simulink model "acf_force_control_fixed_upper_20261005"  (R2026b)
settings: Solver=ode4  StopTime=2  FixedStep=3.3333333333333333e-06
PostLoadFcn:
  | addpath(fullfile(fileparts(get_param(bdroot,'FileName')),'helpers'));
InitFcn:
  | acf_fixed_apply(bdroot);
model workspace (MAT data in the model file):
  p : object (value not decoded)
  pCompliant : object (value not decoded)
  pDefault : object (value not decoded)
symbols that are objects in the model workspace (value not decoded): p
undefined symbols (not defined in the file or in its folder): DiscIntNeverNeededParam
(part 1 of 3)
settings Model: Creator=tommie  LastModifiedBy=tommie
settings DataIOCC: SignalLogging=off
settings DebuggingCC: AlgebraicLoopMsg=error
settings RTWCC: GenCodeOnly=on
settings GRTTargetCC: MatFileLogging=off

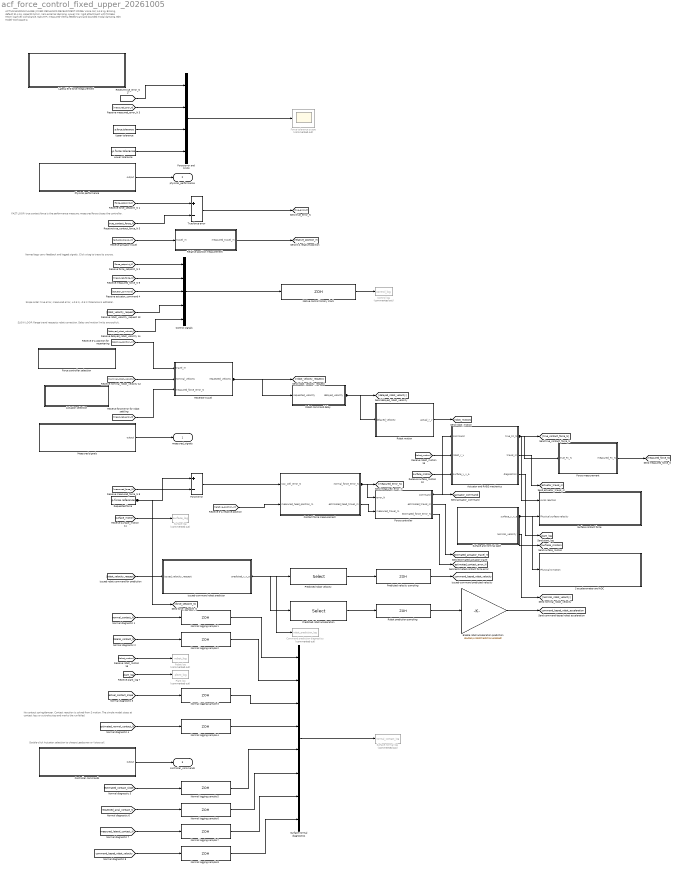
== system acf_force_control_fixed_upper_20261005 ==
  note: FAST LOOP: true contact force is the performance measure; measured force closes the controller.
  note: SLOW LOOP: flange travel requests robot correction. Delay and motion limits are explicit.
  note: No contact spring/damper. Contact reaction is solved from S motion.
      | The simple model stops at contact loss or a stroke stop and marks the run failed.
  note: Scope order: true error, measured error, +0.5 N, -0.5 N (tolerance is editable).
  note: Double-click Actuator selection to choose Leadscrew or Voice coil.
  note: Named tags carry feedback and logged signals. Click a tag to trace its source.
  note: ACTIVE SANDING FLANGE | FIXED MECHANICS DEVELOPMENT MODEL
      | Voice coil; A1.5 kg, B0.6 kg, default S1.4 kg. Upper20 N/mm, zero external damping.
      | Lower link: rigid attachment with finite64 MN/m load-cell compliance.
      | Native PI, measured-inertia feedforward and bounded modal damping. Edit Model Workspace p.
  Actuator and RABS mechanics : Subsystem
  Actuator selection : Subsystem  mask(Active contact flange actuator selection){ActuatorChoice=Voice coil}
      mask prompts: ActuatorChoice "Actuator"
      mask help: Choose the motor before running. Mechanical, surface and sensor settings are preserved. Force-controller gains, command units and initial holding current are recalculated for the selected drive.
      mask TypeOptions ActuatorChoice: Leadscrew | Voice coil | Ideal position (reference)
      mask Callback ActuatorChoice: acf_fixed_select_actuator(bdroot(gcb),get_param(gcb,'ActuatorChoice'));
      mask Display: disp(sprintf('Actuator selection\n%s',get_param(gcb,'ActuatorChoice')));
  Command prediction diagnostics : ToWorkspace  Commented=on  VariableName=robot_prediction_log  SaveFormat=Timeseries  SampleTime=p.sim.step
  Contact force measurement : Subsystem
  Control log : ToWorkspace  Commented=on  VariableName=control_log  SaveFormat=Timeseries  SampleTime=p.sim.step
  Control signals : Mux  Inputs=5
  Controller commands : Subsystem
  Enable robot acceleration prediction : Gain  Gain=double(p.robotPrediction.enabled)
  Force controller : Subsystem  Variant=on  VariantControlMode=label  LabelModeActiveChoice=Coil PI and PID
  Force controller selection : Subsystem  mask{ControllerChoice=PI, AccelerationFeedforward=on}
      mask prompts: ControllerChoice "Voice-coil control strategy"; AccelerationFeedforward "Measured acceleration feedforward"
      mask help: Native force/stroke observer or conventional force PI/PID. Gains remain editable in the Model Workspace p. The saved recommended preset includes the qualified upper-rigid PID gains.
      mask TypeOptions ControllerChoice: PI | PID
      mask Callback ControllerChoice: acf_fixed_select_controller(bdroot);
      mask Callback AccelerationFeedforward: acf_fixed_select_controller(bdroot(gcb));
      mask Display: disp('Choose coil controller')
  Force error : Sum  Inputs=+-
  Force error and limits : Mux
  Force measurement : Subsystem
  Force tolerance scope : Scope  Commented=on
  Issued-command robot predictor : Subsystem
  Lateral B-S force measurement : Subsystem
  Lower tolerance : Constant  Value=-p.force.tolerance
  Measured signals : Subsystem
  Native control history clock : ZeroOrderHold  SampleTime=p.sim.step
  Normal logging sample {1..8} (8 alike) : ZeroOrderHold  SampleTime=p.sim.step
  Physical performance : Subsystem
  Plant log : ToWorkspace  Commented=on  VariableName=plant_log  SaveFormat=Timeseries  SampleTime=p.sim.step
  Predicted robot acceleration : Selector  InputPortWidth=3  IndexOptions=Index vector (dialog)  Indices=3  OutputSizes=1
  Predicted robot velocity : Selector  InputPortWidth=3  IndexOptions=Index vector (dialog)  Indices=2  OutputSizes=1
  Predicted velocity sampling : ZeroOrderHold  SampleTime=p.force.sampleTime
  Recenter travel : Subsystem
  Relative position measurement : Subsystem
  Requested force : Constant  Value=p.force.reference
  Robot command delay : Subsystem
  Robot log : ToWorkspace  Commented=on  VariableName=robot_log  SaveFormat=Timeseries  SampleTime=p.sim.step
  Robot motion : Subsystem
  Robot prediction sampling : ZeroOrderHold  SampleTime=p.force.sampleTime
  S accelerometer and ADC : Subsystem
  Surface and nominal path : Subsystem
  Surface contact force : Subsystem
  Surface log : ToWorkspace  Commented=on  VariableName=surface_log  SaveFormat=Timeseries  SampleTime=p.sim.step
  Surface normal diagnostics : Mux  Inputs=8
  Surface normal log : ToWorkspace  Commented=on  VariableName=normal_contact_log  SaveFormat=Timeseries  SampleTime=p.sim.step
  True force error : Sum  Inputs=+-
  Upper tolerance : Constant  Value=p.force.tolerance
  measured_signals : Outport
  physical_performance : Outport  Port=2
  controller_commands : Outport  Port=3
  tag scope: command_based_robot_acceleration=global, command_based_robot_velocity=global, estimated_actuator_travel_m=global, estimated_contact_error_N=global, plant_log=global, surface_motion=global
  wires:
  Force measurement/1(measured_Fc_N) -> [measured_force_N]
  Enable robot acceleration prediction/1 -> [command_based_robot_acceleration]
  Surface and nominal path/1(surface_y_v_a) -> S accelerometer and ADC/1(Physical S motion), Surface contact force/2(Physical surface velocity), [surface_motion]
  Surface and nominal path/2(nominal_velocity) -> [nominal_robot_velocity]
  Actuator and RABS mechanics/3(diagnostics) -> [plant_log]
  Actuator and RABS mechanics/1(true_Fc_N) -> Surface contact force/1(Axial reaction), [true_contact_force_N], Force measurement/1(true_Fc_N)
  Robot prediction sampling/1 -> Enable robot acceleration prediction/1
  Predicted velocity sampling/1 -> [command_based_robot_velocity]
  Force controller/3(estimated_force_error_N) -> [estimated_contact_error_N]
  Force controller/2(estimated_travel_m) -> [estimated_actuator_travel_m]
  Controller commands/1(output) -> controller_commands/1
  [actual_contact_slope] -> Normal logging sample 3/1
  Predicted robot acceleration/1 -> Robot prediction sampling/1
  Lower tolerance/1 -> Force error and limits/4
  Force error/1 -> Contact force measurement/1(raw_cell_error_N)
  [relative_position_m] -> Contact force measurement/2(measured_head_position_m)
  [normal_contact_N] -> Normal logging sample 1/1
  [measured_force_N] -> Force error/2
  [command_based_robot_velocity] -> Normal logging sample 8/1
  [estimated_contact_slope] -> Normal logging sample 5/1
  Recenter travel/1(requested_velocity) -> [robot_velocity_request], Robot command delay/1(requested_velocity)
  Requested force/1 -> [force_setpoint_N], Force error/1
  [robot_velocity_request] -> Issued-command robot predictor/1(issued_velocity_request)
  [robot_velocity_request] -> Control signals/4
  [relative_position_m] -> Recenter travel/1(travel_m)
  [measured_error_N] -> Force error and limits/2
  [measured_lateral_contact_N] -> Normal logging sample 7/1
  Issued-command robot predictor/1(predicted_r_v_a) -> Predicted robot velocity/1, Command prediction diagnostics/1, Predicted robot acceleration/1
  [actuator_command] -> Control signals/3
  Measured signals/1(output) -> measured_signals/1
  Physical performance/1(output) -> physical_performance/1
  [estimated_normal_contact_N] -> Normal logging sample 4/1
  [plant_log] -> Plant log/1
  [measured_error_N] -> Recenter travel/3(measured_force_error_N)
  Robot command delay/1(delayed_velocity) -> [delayed_robot_velocity], Robot motion/1(delayed_velocity)
  [force_setpoint_N] -> True force error/1
  [true_error_N] -> Force error and limits/1
  Robot motion/1(actual_r_v) -> [robot_motion]
  Normal logging sample 8/1 -> Surface normal diagnostics/8
  Upper tolerance/1 -> Force error and limits/3
  [true_contact_force_N] -> True force error/2
  [surface_motion] -> Actuator and RABS mechanics/3(surface_y_v_a)
  Normal logging sample 5/1 -> Surface normal diagnostics/5
  [delayed_robot_velocity] -> Control signals/5
  [measured_force_N] -> Control signals/2
  Normal logging sample 3/1 -> Surface normal diagnostics/3
  Contact force measurement/2(estimated_head_travel_m) -> Force controller/2(measured_travel_m)
  [nominal_robot_velocity] -> Recenter travel/2(nominal_velocity)
  [requested_axial_contact_N] -> Normal logging sample 6/1
  Relative position measurement/1(measured_travel_m) -> [relative_position_m]
  Control signals/1 -> Native control history clock/1
  Force error and limits/1 -> Force tolerance scope/1
  [actuator_travel_m] -> Relative position measurement/1(travel_m)
  Force controller/1(command) -> [actuator_command], Actuator and RABS mechanics/1(command)
  True force error/1 -> [true_error_N]
  [robot_motion] -> Robot log/1
  Normal logging sample 1/1 -> Surface normal diagnostics/1
  Normal logging sample 2/1 -> Surface normal diagnostics/2
  Normal logging sample 4/1 -> Surface normal diagnostics/4
  Normal logging sample 6/1 -> Surface normal diagnostics/6
  Actuator and RABS mechanics/2(travel_m) -> [actuator_travel_m]
  Normal logging sample 7/1 -> Surface normal diagnostics/7
  [surface_motion] -> Surface log/1
  Contact force measurement/1(normal_force_error_N) -> [measured_error_N], Force controller/1(error_N)
  Predicted robot velocity/1 -> Predicted velocity sampling/1
  [lateral_contact_N] -> Normal logging sample 2/1
  Surface normal diagnostics/1 -> Surface normal log/1
  [force_setpoint_N] -> Control signals/1
  Native control history clock/1 -> Control log/1
  [robot_motion] -> Actuator and RABS mechanics/2(robot_r_v)

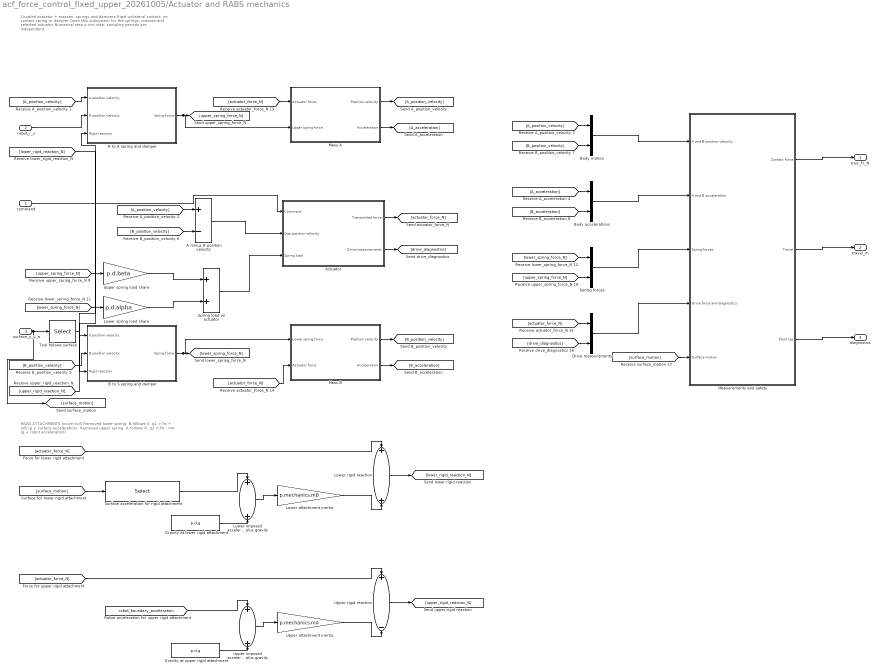
== system acf_force_control_fixed_upper_20261005/Actuator and RABS mechanics ==
  note: Coupled actuator + masses, springs and dampers
      | Rigid unilateral contact; no contact spring or damper
      | Open this subsystem for the springs, masses and selected actuator
      | Numerical step p.sim.step; sampling periods are independent.
  note: RIGID ATTACHMENTS (voice coil)
      | Removed lower spring: B follows S, q1 = Fa + mB (g + surface acceleration).
      | Removed upper spring: A follows R, q2 = Fa - mA (g + robot acceleration).
  command : Inport
  robot_r_v : Inport  Port=2
  surface_y_v_a : Inport  Port=3
  A minus B position velocity : Sum  Inputs=+-
  Actuator : Subsystem  Variant=on  VariantControlMode=label  LabelModeActiveChoice=Voice coil
  B to S spring and damper : Subsystem
  Body accelerations : Mux  Inputs=2
  Body motion : Mux  Inputs=2
  Drive measurements : Mux  Inputs=2
  Gravity at lower rigid attachment : Constant  Value=p.d.g
  Gravity at upper rigid attachment : Constant  Value=p.d.g
  Lower attachment inertia : Gain  Gain=p.mechanics.mB
  Lower imposed acceleration plus gravity : Sum
  Lower rigid reaction : Sum
  Lower spring load share : Gain  Gain=p.d.alpha
  Mass A : Subsystem
  Mass B : Subsystem
  Measurements and safety : Subsystem
  R to A spring and damper : Subsystem
  Spring forces : Mux  Inputs=2
  Spring load on actuator : Sum
  Surface acceleration for rigid attachment : Selector  InputPortWidth=3  IndexOptions=Index vector (dialog)  Indices=3  OutputSizes=1
  Tool follows surface : Selector  InputPortWidth=3  IndexOptions=Index vector (dialog)  Indices=[1 2]  OutputSizes=1
  Upper attachment inertia : Gain  Gain=p.mechanics.mA
  Upper imposed acceleration plus gravity : Sum
  Upper rigid reaction : Sum  Inputs=+-
  Upper spring load share : Gain  Gain=p.d.beta
  true_Fc_N : Outport
  travel_m : Outport  Port=2
  diagnostics : Outport  Port=3
  wires:
  [A_position_velocity] -> A minus B position velocity/1
  [B_position_velocity] -> A minus B position velocity/2
  command/1 -> Actuator/1(Command)
  A minus B position velocity/1 -> Actuator/2(Gap position velocity)
  Spring load on actuator/1 -> Actuator/3(Spring load)
  Tool follows surface/1 -> B to S spring and damper/1(S position velocity)
  [B_position_velocity] -> B to S spring and damper/2(B position velocity)
  [A_acceleration] -> Body accelerations/1
  [B_acceleration] -> Body accelerations/2
  [A_position_velocity] -> Body motion/1
  [B_position_velocity] -> Body motion/2
  [actuator_force_N] -> Drive measurements/1
  [drive_diagnostics] -> Drive measurements/2
  [lower_spring_force_N] -> Lower spring load share/1
  [actuator_force_N] -> Mass A/1(Actuator force)
  R to A spring and damper/1(Spring force) -> Mass A/2(Upper spring force), [upper_spring_force_N]
  B to S spring and damper/1(Spring force) -> Mass B/1(Lower spring force), [lower_spring_force_N]
  [actuator_force_N] -> Mass B/2(Actuator force)
  Body motion/1 -> Measurements and safety/1(A and B position velocity)
  Body accelerations/1 -> Measurements and safety/2(A and B acceleration)
  Spring forces/1 -> Measurements and safety/3(Spring forces)
  Drive measurements/1 -> Measurements and safety/4(Drive force and diagnostics)
  [surface_motion] -> Measurements and safety/5(Surface motion)
  [A_position_velocity] -> R to A spring and damper/1(A position velocity)
  robot_r_v/1 -> R to A spring and damper/2(R position velocity)
  Mass A/2(Acceleration) -> [A_acceleration]
  Mass A/1(Position velocity) -> [A_position_velocity]
  Mass B/2(Acceleration) -> [B_acceleration]
  Mass B/1(Position velocity) -> [B_position_velocity]
  Actuator/1(Transmitted force) -> [actuator_force_N]
  Actuator/2(Drive measurements) -> [drive_diagnostics]
  surface_y_v_a/1 -> [surface_motion], Tool follows surface/1
  [lower_spring_force_N] -> Spring forces/1
  [upper_spring_force_N] -> Spring forces/2
  Upper spring load share/1 -> Spring load on actuator/1
  Lower spring load share/1 -> Spring load on actuator/2
  [upper_spring_force_N] -> Upper spring load share/1
  Measurements and safety/1(Contact force) -> true_Fc_N/1
  Measurements and safety/2(Travel) -> travel_m/1
  Measurements and safety/3(Plant log) -> diagnostics/1
  [actuator_force_N] -> Lower rigid reaction/1
  [surface_motion] -> Surface acceleration for rigid attachment/1
  Surface acceleration for rigid attachment/1 -> Lower imposed acceleration plus gravity/1
  Gravity at lower rigid attachment/1 -> Lower imposed acceleration plus gravity/2
  Lower imposed acceleration plus gravity/1 -> Lower attachment inertia/1
  Lower attachment inertia/1 -> Lower rigid reaction/2
  Lower rigid reaction/1 -> [lower_rigid_reaction_N]
  [actuator_force_N] -> Upper rigid reaction/1
  [robot_boundary_acceleration] -> Upper imposed acceleration plus gravity/1
  Gravity at upper rigid attachment/1 -> Upper imposed acceleration plus gravity/2
  Upper imposed acceleration plus gravity/1 -> Upper attachment inertia/1
  Upper attachment inertia/1 -> Upper rigid reaction/2
  Upper rigid reaction/1 -> [upper_rigid_reaction_N]
  [lower_rigid_reaction_N] -> B to S spring and damper/3(Rigid reaction)
  [upper_rigid_reaction_N] -> R to A spring and damper/3(Rigid reaction)

== system acf_force_control_fixed_upper_20261005/Actuator selection ==

== system acf_force_control_fixed_upper_20261005/Contact force measurement ==
  raw_cell_error_N : Inport
  measured_head_position_m : Inport  Port=2
  Contact force reconstruction : Subsystem
  Head motion estimator : Subsystem
  Normal force error sign : Gain  Gain=-1
  Normal force projection : Subsystem
  normal_force_error_N : Outport
  estimated_head_travel_m : Outport  Port=2
  tag scope: inertial_axial_reference_deviation_N=global, inertial_head_gap_velocity=global
  wires:
  raw_cell_error_N/1 -> Contact force reconstruction/1(raw_cell_error_N)
  measured_head_position_m/1 -> Head motion estimator/1(measured_head_position_m)
  Contact force reconstruction/1(axial_contact_N) -> Normal force projection/1(Compensated axial force)
  Contact force reconstruction/2(lateral_contact_N) -> Normal force projection/2(Compensated lateral force)
  Head motion estimator/1(head_gap_velocity_m_s) -> Normal force projection/3(Head gap velocity), [inertial_head_gap_velocity]
  Head motion estimator/2(estimated_head_travel_m) -> estimated_head_travel_m/1
  Normal force projection/1(normal_force_deviation_N) -> Normal force error sign/1
  Normal force error sign/1 -> normal_force_error_N/1
  Normal force projection/2(axial_reference_deviation_N) -> [inertial_axial_reference_deviation_N]
  Contact force reconstruction/3(measured_lower_force_deviation_N) -> Head motion estimator/2(Measured lower force deviation)

== system acf_force_control_fixed_upper_20261005/Controller commands ==
  Double 1 : DataTypeConversion  OutDataTypeStr=double  SaturateOnIntegerOverflow=off  RndMeth=Floor
  Double 2 : DataTypeConversion  OutDataTypeStr=double  SaturateOnIntegerOverflow=off  RndMeth=Floor
  Double 3 : DataTypeConversion  OutDataTypeStr=double  SaturateOnIntegerOverflow=off  RndMeth=Floor
  Vector : Mux  Inputs=3
  output : Outport
  wires:
  [rl_baseline_current] -> Double 1/1
  Double 1/1 -> Vector/1
  [rl_baseline_robot] -> Double 2/1
  Double 2/1 -> Vector/2
  [rl_equilibrium_current] -> Double 3/1
  Double 3/1 -> Vector/3
  Vector/1 -> output/1

== system acf_force_control_fixed_upper_20261005/Force controller ==
  error_N : Inport
  measured_travel_m : Inport  Port=2
  Coil PI and PID : Subsystem  VariantControl=Coil PI and PID
  Drive PI and PID : Subsystem  VariantControl=Drive PI and PID
  command : Outport
  estimated_travel_m : Outport  Port=2
  estimated_force_error_N : Outport  Port=3

== system acf_force_control_fixed_upper_20261005/Force controller selection ==

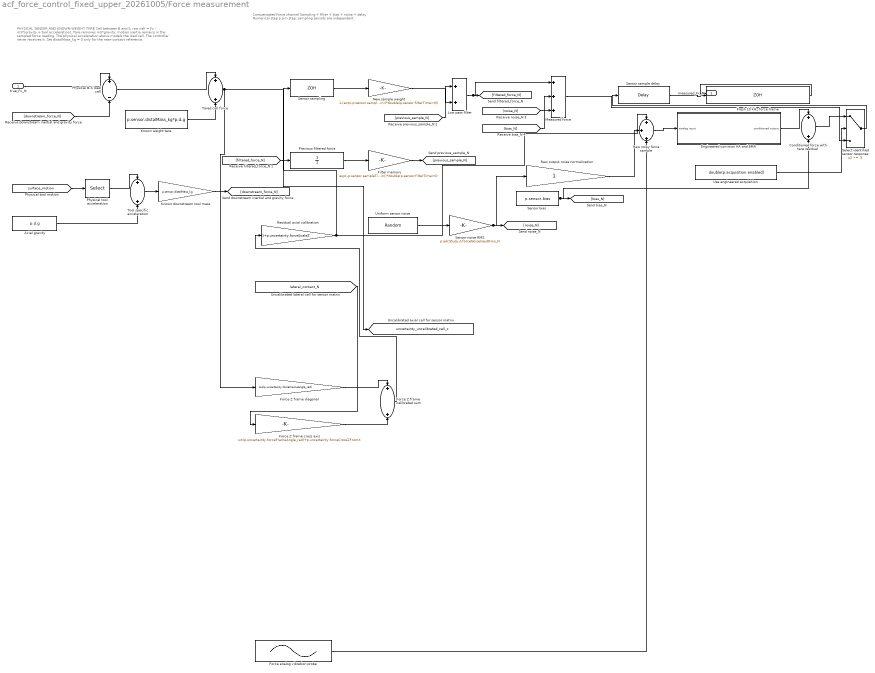
== system acf_force_control_fixed_upper_20261005/Force measurement ==
  note: Compensated force channel
      | Sampling + filter + bias + noise + delay
      | Numerical step p.sim.step; sampling periods are independent.
  note: PHYSICAL SENSOR AND KNOWN-WEIGHT TARE
      | Cell between B and S: raw cell = Fc - mS*(gravity + tool acceleration).
      | Tare removes mS*gravity; motion inertia remains in the sampled force reading.
      | The physical acceleration above models the load cell. The controller never receives it.
      | Set distalMass_kg = 0 only for the near-contact reference.
  true_Fc_N : Inport
  Axial gravity : Constant  Value=p.d.g
  Conditioned force with tare residual : Sum
  Engineered common AA and EMA : Subsystem
  Filter memory : Gain  Gain=exp(-p.sensor.sampleTime/max(p.sensor.filterTime,realmin))*double(p.sensor.filterTime>0)
  Force Z frame calibrated sum : Sum
  Force Z frame cross axis : Gain  Gain=sin(p.uncertainty.forceFrameAngle_rad)+p.uncertainty.forceCrossZFromX
  Force Z frame diagonal : Gain  Gain=cos(p.uncertainty.forceFrameAngle_rad)
  Force analog vibration probe : Sin  Amplitude=p.adcStudy.forceAnalogToneAmplitude_N  Frequency=2*pi*p.adcStudy.analogToneFrequency_Hz  Phase=p.adcStudy.analogTonePhase_rad  SampleTime=0
  Fresh 10 kHz force frame : ZeroOrderHold  SampleTime=p.force.sampleTime
  Known downstream tool mass : Gain  Gain=p.sensor.distalMass_kg
  Known weight tare : Constant  Value=p.sensor.distalMass_kg*p.d.g
  Low pass filter : Sum
  Measured force : Sum  Inputs=+++
  New sample weight : Gain  Gain=1-(exp(-p.sensor.sampleTime/max(p.sensor.filterTime,realmin))*double(p.sensor.filterTime>0))
  Physical B-S load cell : Sum  Inputs=+-
  Physical tool acceleration : Selector  InputPortWidth=3  IndexOptions=Index vector (dialog)  Indices=3  OutputSizes=1
  Previous filtered force : UnitDelay  InitialCondition=p.force.reference*(1+p.uncertainty.forceScaleZ)*(cos(p.uncertainty.forceFrameAngle_rad)-p.contact.mu*(sin(p.uncertainty.forceFrameAngle_rad)+p.uncertainty.forceCrossZFromX))  SampleTime=p.sensor.sampleTime
  Raw noisy force sample : Sum  Inputs=+++
  Raw output-noise normalization : Gain
  Residual axial calibration : Gain  Gain=1+p.uncertainty.forceScaleZ
  Select identified sensor response : Switch  Threshold=.5  SaturateOnIntegerOverflow=off  InputSameDT=off
  Sensor bias : Constant  Value=p.sensor.bias
  Sensor noise RMS : Gain  Gain=p.adcStudy.d.forceNoiseInputRms_N
  Sensor sample delay : TransportDelay  DelayTime=p.adcStudy.d.channels.force.pipelineDelay_s  InitialOutput=round((((p.force.reference*(1+p.uncertainty.forceScaleZ)*(cos(p.uncertainty.forceFrameAngle_rad)-p.contact.mu*(sin(p.uncertainty.forceFrameAngle_rad)+p.uncertainty.forceCrossZFromX))))+(p.adcStudy.d.forceGravityOffset_N))/(max(p.adcStudy.forceQuantum_N,1e-15)))*(max(p.adcStudy.forceQuantum_N,1e-15))-round((p.adcStudy.d.forceGravityOffset_N)/(max(p.adcStudy.forceQuantum_N,1e-15)))*(max(p.adcStudy.forceQuantum_N,1e-15))+(p.sensor.bias)
  Sensor sampling : ZeroOrderHold  SampleTime=p.sensor.sampleTime
  Tared cell force : Sum
  Tool specific acceleration : Sum
  Uniform sensor noise : UniformRandomNumber  Minimum=-sqrt(3)  Maximum=sqrt(3)  Seed=p.sensor.seed  SampleTime=p.sensor.sampleTime
  Use engineered acquisition : Constant  Value=double(p.acquisition.enabled)
  measured_Fc_N : Outport
  tag scope: uncertainty_uncalibrated_cell_z=global
  wires:
  Previous filtered force/1 -> Filter memory/1
  [previous_sample_N] -> Low pass filter/1
  New sample weight/1 -> Low pass filter/2
  Low pass filter/1 -> Measured force/1, [filtered_force_N]
  [bias_N] -> Measured force/2
  [noise_N] -> Measured force/3
  Sensor sampling/1 -> New sample weight/1
  [filtered_force_N] -> Previous filtered force/1
  Sensor bias/1 -> [bias_N], Conditioned force with tare residual/2
  Sensor noise RMS/1 -> [noise_N], Raw output-noise normalization/1
  Filter memory/1 -> [previous_sample_N]
  Uniform sensor noise/1 -> Sensor noise RMS/1
  Measured force/1 -> Select identified sensor response/3
  true_Fc_N/1 -> Physical B-S load cell/1
  [downstream_force_N] -> Physical B-S load cell/2
  Physical B-S load cell/1 -> Tared cell force/1
  Known weight tare/1 -> Tared cell force/2
  [surface_motion] -> Physical tool acceleration/1
  Physical tool acceleration/1 -> Tool specific acceleration/1
  Axial gravity/1 -> Tool specific acceleration/2
  Tool specific acceleration/1 -> Known downstream tool mass/1
  Known downstream tool mass/1 -> [downstream_force_N]
  Raw output-noise normalization/1 -> Raw noisy force sample/2
  Conditioned force with tare residual/1 -> Select identified sensor response/1
  Use engineered acquisition/1 -> Select identified sensor response/2
  Fresh 10 kHz force frame/1 -> measured_Fc_N/1
  Tared cell force/1 -> [uncertainty_uncalibrated_cell_z], Force Z frame diagonal/1
  Residual axial calibration/1 -> Sensor sampling/1, Raw noisy force sample/1
  [lateral_contact_N] -> Force Z frame cross axis/1
  Force Z frame diagonal/1 -> Force Z frame calibrated sum/1
  Force Z frame cross axis/1 -> Force Z frame calibrated sum/2
  Force Z frame calibrated sum/1 -> Residual axial calibration/1
  Force analog vibration probe/1 -> Raw noisy force sample/3
  Raw noisy force sample/1 -> Engineered common AA and EMA/1(analog input)
  Engineered common AA and EMA/1(conditioned output) -> Conditioned force with tare residual/1
  Select identified sensor response/1 -> Sensor sample delay/1
  Sensor sample delay/1 -> Fresh 10 kHz force frame/1

== system acf_force_control_fixed_upper_20261005/Issued-command robot predictor ==
  issued_velocity_request : Inport
  Expected acceleration limit : Saturate  UpperLimit=p.robotPrediction.maxAcceleration  LowerLimit=-p.robotPrediction.maxAcceleration
  Expected command delay : Delay  DelayLengthSource=Input port  DelayLength=p.robotPrediction.delaySamples  DelayLengthUpperLimit=12  InitialCondition=p.robot.nominalVelocity*double(~p.robotPrediction.boundedNominalPath)  PreventDirectFeedthrough=on  DiagnosticForDelayLength=Error  UseCircularBuffer=on  SampleTime=p.robot.sampleTime
      settings: InputPortMap=u0,p1
  Expected speed limit : Saturate  UpperLimit=p.robotPrediction.maxSpeed  LowerLimit=-p.robotPrediction.maxSpeed
  Expected velocity response : Gain  Gain=1/p.robotPrediction.responseTime
  Predicted position velocity acceleration : Mux  Inputs=3
  Predicted relative position : Integrator
  Predicted velocity : Integrator
  Predicted velocity error : Sum  Inputs=+-
  RL reset-fixed queue length : Constant  Value=p.robotPrediction.delaySamples
  predicted_r_v_a : Outport
  wires:
  Predicted position velocity acceleration/1 -> predicted_r_v_a/1
  Predicted relative position/1 -> Predicted position velocity acceleration/1
  Predicted velocity/1 -> Predicted position velocity acceleration/2, Predicted relative position/1, [prediction_internal_velocity]
  Expected acceleration limit/1 -> Predicted position velocity acceleration/3, Predicted velocity/1
  Expected velocity response/1 -> Expected acceleration limit/1
  Predicted velocity error/1 -> Expected velocity response/1
  [prediction_internal_velocity] -> Predicted velocity error/2
  Expected speed limit/1 -> Predicted velocity error/1
  Expected command delay/1 -> Expected speed limit/1
  issued_velocity_request/1 -> Expected command delay/1
  RL reset-fixed queue length/1 -> Expected command delay/2

== system acf_force_control_fixed_upper_20261005/Lateral B-S force measurement ==
  Conditioned force with tare residual : Sum
  Engineered common AA and EMA : Subsystem
  Filter memory : UnitDelay  InitialCondition=p.force.reference*(1+p.uncertainty.forceScaleX)*(-p.contact.mu*cos(p.uncertainty.forceFrameAngle_rad)-sin(p.uncertainty.forceFrameAngle_rad)+p.uncertainty.forceCrossXFromZ)  SampleTime=p.sensor.sampleTime
  Filtered derivative memory : Gain  Gain=exp(-p.sensor.sampleTime/p.contact.lateralDerivativeFilterTime_s)
  Filtered derivative new sample : Gain  Gain=(1-exp(-p.sensor.sampleTime/p.contact.lateralDerivativeFilterTime_s))/p.sensor.sampleTime
  Filtered lateral force derivative : Sum
  Force X frame calibrated sum : Sum
  Force X frame cross axis : Gain  Gain=-sin(p.uncertainty.forceFrameAngle_rad)+p.uncertainty.forceCrossXFromZ
  Force X frame diagonal : Gain  Gain=cos(p.uncertainty.forceFrameAngle_rad)
  Fresh 10 kHz force frame : ZeroOrderHold  SampleTime=p.force.sampleTime
  Identified lateral latency : Gain  Gain=p.contact.lateralPredictionTime_s
  Independent lateral noise : UniformRandomNumber  Minimum=-sqrt(3)  Maximum=sqrt(3)  Seed=p.sensor.seed+197  SampleTime=p.sensor.sampleTime
  Known tare residual bias : Constant  Value=p.contact.lateralBias_N
  Lateral analog vibration probe : Sin  Amplitude=p.adcStudy.lateralAnalogToneAmplitude_N  Frequency=2*pi*p.adcStudy.analogToneFrequency_Hz  Phase=p.adcStudy.analogTonePhase_rad  SampleTime=0
  Measured lateral force increment : Sum  Inputs=+-
  New sample weight : Gain  Gain=1-exp(-p.sensor.sampleTime/max(p.sensor.filterTime,realmin))*double(p.sensor.filterTime>0)
  Noise RMS : Gain  Gain=p.adcStudy.d.lateralNoiseInputRms_N
  Noisy tared lateral force : Sum  Inputs=+++
  Old sample weight : Gain  Gain=exp(-p.sensor.sampleTime/max(p.sensor.filterTime,realmin))*double(p.sensor.filterTime>0)
  Present lateral force estimate : Sum
  Previous lateral derivative : UnitDelay  SampleTime=p.sensor.sampleTime
  Previous measured lateral force : UnitDelay  InitialCondition=p.force.reference*(1+p.uncertainty.forceScaleX)*(-p.contact.mu*cos(p.uncertainty.forceFrameAngle_rad)-sin(p.uncertainty.forceFrameAngle_rad)+p.uncertainty.forceCrossXFromZ)+p.contact.lateralBias_N  SampleTime=p.sensor.sampleTime
  Raw noisy force sample : Sum  Inputs=+++
  Raw output-noise normalization : Gain
  Residual lateral calibration : Gain  Gain=1+p.uncertainty.forceScaleX
  Select identified sensor response : Switch  Threshold=.5  SaturateOnIntegerOverflow=off  InputSameDT=off
  Sensor low pass : Sum
  Sensor sample delay : TransportDelay  DelayTime=p.adcStudy.d.channels.lateral.pipelineDelay_s  InitialOutput=round((((p.force.reference*(1+p.uncertainty.forceScaleX)*(-p.contact.mu*cos(p.uncertainty.forceFrameAngle_rad)-sin(p.uncertainty.forceFrameAngle_rad)+p.uncertainty.forceCrossXFromZ)))+(p.adcStudy.d.lateralGravityOffset_N))/(max(p.adcStudy.forceQuantum_N,1e-15)))*(max(p.adcStudy.forceQuantum_N,1e-15))-round((p.adcStudy.d.lateralGravityOffset_N)/(max(p.adcStudy.forceQuantum_N,1e-15)))*(max(p.adcStudy.forceQuantum_N,1e-15))+(p.contact.lateralBias_N)
  Sensor sampling : ZeroOrderHold  SampleTime=p.sensor.sampleTime
  Use engineered acquisition : Constant  Value=double(p.acquisition.enabled)
  tag scope: measured_lateral_contact_N=global, predicted_lateral_contact_N=global
  wires:
  Sensor sampling/1 -> New sample weight/1
  New sample weight/1 -> Sensor low pass/1
  Sensor low pass/1 -> Filter memory/1, Noisy tared lateral force/1
  Filter memory/1 -> Old sample weight/1
  Old sample weight/1 -> [normal_lateral_filter_local]
  [normal_lateral_filter_local] -> Sensor low pass/2
  Independent lateral noise/1 -> Noise RMS/1
  Noise RMS/1 -> Noisy tared lateral force/2, Raw output-noise normalization/1
  Known tare residual bias/1 -> Noisy tared lateral force/3, Conditioned force with tare residual/2
  Noisy tared lateral force/1 -> Select identified sensor response/3
  Previous measured lateral force/1 -> Measured lateral force increment/2
  Measured lateral force increment/1 -> Filtered derivative new sample/1
  Filtered derivative new sample/1 -> Filtered lateral force derivative/1
  Filtered lateral force derivative/1 -> Previous lateral derivative/1, Identified lateral latency/1
  Previous lateral derivative/1 -> Filtered derivative memory/1
  Filtered derivative memory/1 -> Filtered lateral force derivative/2
  Identified lateral latency/1 -> Present lateral force estimate/2
  Present lateral force estimate/1 -> [predicted_lateral_contact_N]
  Raw output-noise normalization/1 -> Raw noisy force sample/2
  Conditioned force with tare residual/1 -> Select identified sensor response/1
  Use engineered acquisition/1 -> Select identified sensor response/2
  Fresh 10 kHz force frame/1 -> [measured_lateral_contact_N], Previous measured lateral force/1, Measured lateral force increment/1, Present lateral force estimate/1
  Residual lateral calibration/1 -> Sensor sampling/1, Raw noisy force sample/1
  [lateral_contact_N] -> Force X frame diagonal/1
  [uncertainty_uncalibrated_cell_z] -> Force X frame cross axis/1
  Force X frame diagonal/1 -> Force X frame calibrated sum/1
  Force X frame cross axis/1 -> Force X frame calibrated sum/2
  Force X frame calibrated sum/1 -> Residual lateral calibration/1
  Lateral analog vibration probe/1 -> Raw noisy force sample/3
  Raw noisy force sample/1 -> Engineered common AA and EMA/1(analog input)
  Engineered common AA and EMA/1(conditioned output) -> Conditioned force with tare residual/1
  Select identified sensor response/1 -> Sensor sample delay/1
  Sensor sample delay/1 -> Fresh 10 kHz force frame/1

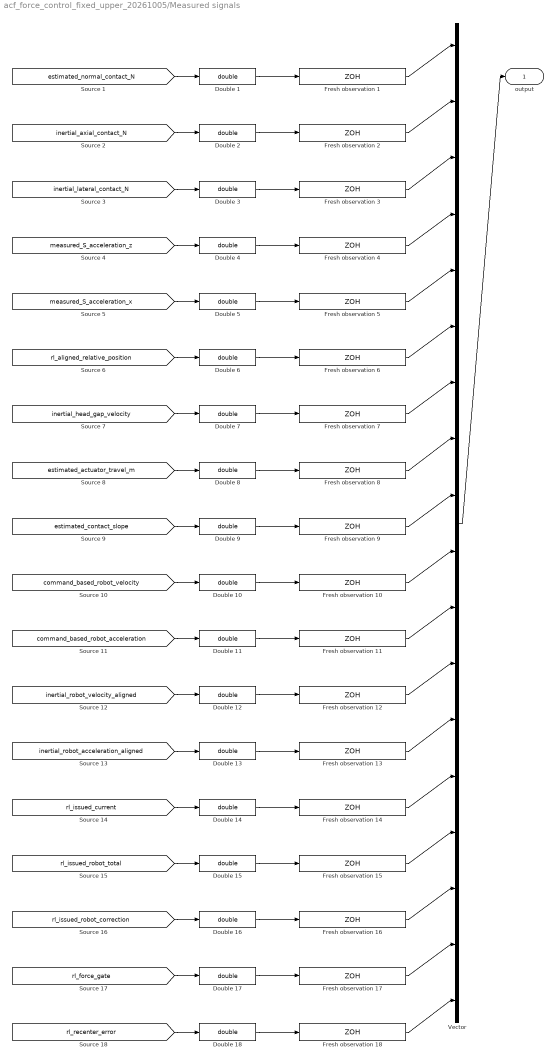
== system acf_force_control_fixed_upper_20261005/Measured signals ==
  Double {1..18} (18 alike) : DataTypeConversion  OutDataTypeStr=double  SaturateOnIntegerOverflow=off  RndMeth=Floor
  Fresh observation {1..18} (18 alike) : ZeroOrderHold  SampleTime=p.force.sampleTime
  Vector : Mux  Inputs=18
  output : Outport
  wires:
  [estimated_normal_contact_N] -> Double 1/1
  Double 1/1 -> Fresh observation 1/1
  Fresh observation 1/1 -> Vector/1
  [inertial_axial_contact_N] -> Double 2/1
  Double 2/1 -> Fresh observation 2/1
  Fresh observation 2/1 -> Vector/2
  [inertial_lateral_contact_N] -> Double 3/1
  Double 3/1 -> Fresh observation 3/1
  Fresh observation 3/1 -> Vector/3
  [measured_S_acceleration_z] -> Double 4/1
  Double 4/1 -> Fresh observation 4/1
  Fresh observation 4/1 -> Vector/4
  [measured_S_acceleration_x] -> Double 5/1
  Double 5/1 -> Fresh observation 5/1
  Fresh observation 5/1 -> Vector/5
  [rl_aligned_relative_position] -> Double 6/1
  Double 6/1 -> Fresh observation 6/1
  Fresh observation 6/1 -> Vector/6
  [inertial_head_gap_velocity] -> Double 7/1
  Double 7/1 -> Fresh observation 7/1
  Fresh observation 7/1 -> Vector/7
  [estimated_actuator_travel_m] -> Double 8/1
  Double 8/1 -> Fresh observation 8/1
  Fresh observation 8/1 -> Vector/8
  [estimated_contact_slope] -> Double 9/1
  Double 9/1 -> Fresh observation 9/1
  Fresh observation 9/1 -> Vector/9
  [command_based_robot_velocity] -> Double 10/1
  Double 10/1 -> Fresh observation 10/1
  Fresh observation 10/1 -> Vector/10
  [command_based_robot_acceleration] -> Double 11/1
  Double 11/1 -> Fresh observation 11/1
  Fresh observation 11/1 -> Vector/11
  [inertial_robot_velocity_aligned] -> Double 12/1
  Double 12/1 -> Fresh observation 12/1
  Fresh observation 12/1 -> Vector/12
  [inertial_robot_acceleration_aligned] -> Double 13/1
  Double 13/1 -> Fresh observation 13/1
  Fresh observation 13/1 -> Vector/13
  [rl_issued_current] -> Double 14/1
  Double 14/1 -> Fresh observation 14/1
  Fresh observation 14/1 -> Vector/14
  [rl_issued_robot_total] -> Double 15/1
  Double 15/1 -> Fresh observation 15/1
  Fresh observation 15/1 -> Vector/15
  [rl_issued_robot_correction] -> Double 16/1
  Double 16/1 -> Fresh observation 16/1
  Fresh observation 16/1 -> Vector/16
  [rl_force_gate] -> Double 17/1
  Double 17/1 -> Fresh observation 17/1
  Fresh observation 17/1 -> Vector/17
  [rl_recenter_error] -> Double 18/1
  Double 18/1 -> Fresh observation 18/1
  Fresh observation 18/1 -> Vector/18
  Vector/1 -> output/1

== system acf_force_control_fixed_upper_20261005/Physical performance ==
  Double 1 : DataTypeConversion  OutDataTypeStr=double  SaturateOnIntegerOverflow=off  RndMeth=Floor
  Double 2 : DataTypeConversion  OutDataTypeStr=double  SaturateOnIntegerOverflow=off  RndMeth=Floor
  Double 3 : DataTypeConversion  OutDataTypeStr=double  SaturateOnIntegerOverflow=off  RndMeth=Floor
  Vector : Mux  Inputs=3
  output : Outport
  wires:
  [normal_contact_N] -> Double 1/1
  Double 1/1 -> Vector/1
  [plant_log] -> Double 2/1
  Double 2/1 -> Vector/2
  [actual_contact_slope] -> Double 3/1
  Double 3/1 -> Vector/3
  Vector/1 -> output/1

== system acf_force_control_fixed_upper_20261005/Recenter travel ==
  note: Mid-stroke - actual travel
      | Deadband + slow gain + nominal robot path
      | Numerical step p.sim.step; sampling periods are independent.
  travel_m : Inport
  nominal_velocity : Inport  Port=2
  measured_force_error_N : Inport  Port=3
  Distance from mid stroke : Sum  Inputs=+-
  Force settling gate : Subsystem
  Gate contact or cell error : Switch  Criteria=u2 ~= 0  SaturateOnIntegerOverflow=off  InputSameDT=off
  Hold recentering : Constant  Value=0
  Measured or estimated travel : Switch  Criteria=u2 ~= 0  SaturateOnIntegerOverflow=off  InputSameDT=off
  Mid stroke : Constant  Value=p.mechanics.midTravel
  Nominal path sampling : ZeroOrderHold  SampleTime=p.robot.sampleTime
  Recenter deadband : DeadZone  LowerValue=-p.robot.deadband  UpperValue=p.robot.deadband
  Recenter gain : Gain  Gain=p.uncertainty.recenterGain
  Robot feedback sampling : ZeroOrderHold  SampleTime=p.robot.sampleTime
  Robot speed limits : Saturate  UpperLimit=p.robot.maxSpeed  LowerLimit=-p.robot.maxSpeed
  Robot velocity request : Sum
  Send correction only when settled : Switch  Threshold=.5  SaturateOnIntegerOverflow=off  InputSameDT=off
  Tool sensor needs gap estimate : Constant  Value=p.sensor.positionModel
  Use reconstructed contact error : Constant  Value=double(p.sensor.distalMass_kg>0 && strcmp(p.actuator.kind,'voice_coil') && strcmp(p.coil.strategy,'observer'))
  requested_velocity : Outport
  tag scope: rl_baseline_robot=global, rl_force_gate=global, rl_issued_robot_correction=global, rl_issued_robot_total=global, rl_recenter_error=global
  wires:
  Robot velocity request/1 -> Robot speed limits/1
  Send correction only when settled/1 -> [rl_issued_robot_correction], Robot velocity request/2
  Force settling gate/1(ready) -> [rl_force_gate], Send correction only when settled/2
  Recenter gain/1 -> Send correction only when settled/1, [rl_baseline_robot]
  Gate contact or cell error/1 -> Force settling gate/1(force_error_N)
  Robot speed limits/1 -> [rl_issued_robot_total], requested_velocity/1
  nominal_velocity/1 -> Nominal path sampling/1
  [nominal_velocity] -> Robot velocity request/1
  Tool sensor needs gap estimate/1 -> Measured or estimated travel/2
  Measured or estimated travel/1 -> Robot feedback sampling/1
  [estimated_contact_error_N] -> Gate contact or cell error/1
  Mid stroke/1 -> Distance from mid stroke/1
  Hold recentering/1 -> Send correction only when settled/3
  [estimated_actuator_travel_m] -> Measured or estimated travel/1
  travel_m/1 -> Measured or estimated travel/3
  Robot feedback sampling/1 -> Distance from mid stroke/2
  Nominal path sampling/1 -> [nominal_velocity]
  Distance from mid stroke/1 -> [rl_recenter_error], Recenter deadband/1
  Use reconstructed contact error/1 -> Gate contact or cell error/2
  measured_force_error_N/1 -> Gate contact or cell error/3
  Recenter deadband/1 -> Recenter gain/1

== system acf_force_control_fixed_upper_20261005/Relative position measurement ==
  travel_m : Inport
  Coordinate reference : Constant  Value=p.mechanics.midTravel
  Measurement delay : Gain
  Position calibrated origin : Bias  Bias=p.d.positionMeasurementInitial  SaturateOnIntegerOverflow=off
  Position calibrated zero : Bias  Bias=-p.d.positionMeasurementInitial  SaturateOnIntegerOverflow=off
  Position noise : UniformRandomNumber  Minimum=-sqrt(3)  Maximum=sqrt(3)  Seed=p.sensor.seed+1  SampleTime=p.d.positionSampleTime
  Position noise RMS : Gain  Gain=p.adcStudy.d.positionNoiseInputRms_m
  Position sampling : ZeroOrderHold  SampleTime=p.d.positionSampleTime
  Residual position calibration : Gain  Gain=1+p.uncertainty.positionScale
  Select A and S : Selector  InputPortWidth=25  IndexOptions=Index vector (dialog)  Indices=[5 7]  OutputSizes=1
  Select position instrument : Switch  Criteria=u2 ~= 0  SaturateOnIntegerOverflow=off  InputSameDT=off
  Sensed position : Sum
  Tool S relative to A : Gain  Gain=[-1 1]  Multiplication=Matrix(K*u)
  Tool measurement coordinate : Sum
  Use toolhead position : Constant  Value=p.sensor.positionModel
  measured_travel_m : Outport
  wires:
  [plant_log] -> Select A and S/1
  Select A and S/1 -> Tool S relative to A/1
  Tool S relative to A/1 -> Tool measurement coordinate/1
  Coordinate reference/1 -> Tool measurement coordinate/2
  Tool measurement coordinate/1 -> Select position instrument/1
  Use toolhead position/1 -> Select position instrument/2
  travel_m/1 -> Select position instrument/3
  Position noise/1 -> Position noise RMS/1
  Position noise RMS/1 -> Sensed position/2
  Select position instrument/1 -> Position calibrated zero/1
  Position calibrated zero/1 -> Residual position calibration/1
  Residual position calibration/1 -> Position calibrated origin/1
  Position calibrated origin/1 -> Position sampling/1, Sensed position/1
  Sensed position/1 -> Measurement delay/1
  Measurement delay/1 -> measured_travel_m/1

== system acf_force_control_fixed_upper_20261005/Robot command delay ==
  note: Delay measured in robot command samples
      | Numerical step p.sim.step; sampling periods are independent.
  requested_velocity : Inport
  Held issued command at transport clock : ZeroOrderHold  SampleTime=p.d.actualRobotTransportSampleTime_s
  RL reset-fixed queue length : Constant  Value=p.d.robotDelaySamples
  Robot command samples : Delay  DelayLengthSource=Input port  DelayLength=p.d.robotDelaySamples  DelayLengthUpperLimit=1000  InitialCondition=p.robot.nominalVelocity*double(~p.robotPrediction.boundedNominalPath)  PreventDirectFeedthrough=on  DiagnosticForDelayLength=Error  UseCircularBuffer=on  SampleTime=p.d.actualRobotTransportSampleTime_s
      settings: InputPortMap=u0,p1
  delayed_velocity : Outport
  wires:
  Robot command samples/1 -> delayed_velocity/1
  requested_velocity/1 -> Held issued command at transport clock/1
  Held issued command at transport clock/1 -> Robot command samples/1
  RL reset-fixed queue length/1 -> Robot command samples/2

== system acf_force_control_fixed_upper_20261005/Robot motion ==
  note: Velocity response + speed/acceleration limits
      | Prescribed robot boundary, no robot force input
      | Numerical step p.sim.step; sampling periods are independent.
  delayed_velocity : Inport
  Requested robot speed : Saturate  UpperLimit=p.robot.maxSpeed  LowerLimit=-p.robot.maxSpeed
  Robot acceleration limits : Saturate  UpperLimit=p.robot.maxAcceleration  LowerLimit=-p.robot.maxAcceleration
  Robot position : Integrator  InitialCondition=p.d.r0
  Robot position and velocity : Mux  Inputs=2
  Robot speed error : Sum  Inputs=+-
  Robot velocity : Integrator
  Velocity response : Gain  Gain=1/p.robot.responseTime
  actual_r_v : Outport
  tag scope: robot_boundary_acceleration=global
  wires:
  delayed_velocity/1 -> Requested robot speed/1
  Velocity response/1 -> Robot acceleration limits/1
  Robot velocity/1 -> Robot position/1, [robot_velocity_m_s]
  [robot_position_m] -> Robot position and velocity/1
  [robot_velocity_m_s] -> Robot position and velocity/2
  Requested robot speed/1 -> Robot speed error/1
  [robot_velocity_m_s] -> Robot speed error/2
  Robot acceleration limits/1 -> Robot velocity/1, [robot_boundary_acceleration]
  Robot position/1 -> [robot_position_m]
  Robot speed error/1 -> Velocity response/1
  Robot position and velocity/1 -> actual_r_v/1

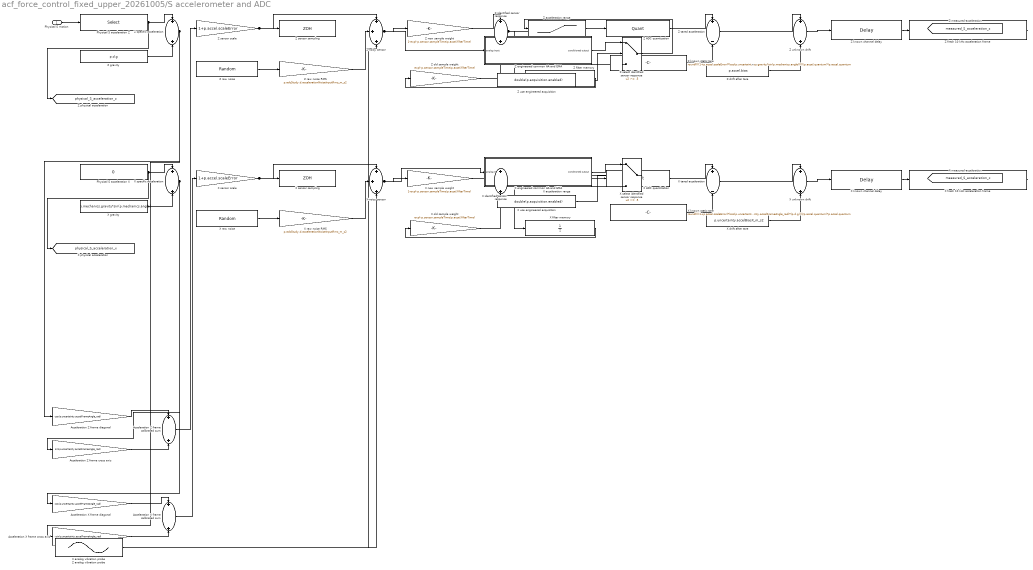
== system acf_force_control_fixed_upper_20261005/S accelerometer and ADC ==
  Physical S motion : Inport
  Acceleration X frame calibrated sum : Sum
  Acceleration X frame cross axis : Gain  Gain=-sin(p.uncertainty.accelFrameAngle_rad)
  Acceleration X frame diagonal : Gain  Gain=cos(p.uncertainty.accelFrameAngle_rad)
  Acceleration Z frame calibrated sum : Sum
  Acceleration Z frame cross axis : Gain  Gain=sin(p.uncertainty.accelFrameAngle_rad)
  Acceleration Z frame diagonal : Gain  Gain=cos(p.uncertainty.accelFrameAngle_rad)
  Physical S acceleration X : Constant  Value=0
  Physical S acceleration Z : Selector  InputPortWidth=3  IndexOptions=Index vector (dialog)  Indices=3  OutputSizes=1
  X ADC quantization : Quantizer  QuantizationInterval=1e-15
  X acceleration range : Saturate  UpperLimit=inf  LowerLimit=-inf
  X analog vibration probe : Sin  Amplitude=p.adcStudy.accelerationXAnalogToneAmplitude_m_s2  Frequency=2*pi*p.adcStudy.analogToneFrequency_Hz  Phase=p.adcStudy.analogTonePhase_rad  SampleTime=0
  X drift after tare : Constant  Value=p.uncertainty.accelBiasX_m_s2
  X engineered common AA and EMA : Subsystem
  X filter memory : UnitDelay  InitialCondition=(1+p.accel.scaleError)*(cos(p.uncertainty.accelFrameAngle_rad)*(p.mechanics.gravity*sin(p.mechanics.angle))-sin(p.uncertainty.accelFrameAngle_rad)*(p.d.g))  SampleTime=p.sensor.sampleTime
  X fresh 10 kHz acceleration frame : ZeroOrderHold  SampleTime=p.force.sampleTime
  X gravity : Constant  Value=p.mechanics.gravity*sin(p.mechanics.angle)
  X identified sensor response : Sum
  X known channel delay : TransportDelay  DelayTime=p.adcStudy.d.channels.acceleration.pipelineDelay_s  InitialOutput=p.uncertainty.accelBiasX_m_s2
  X known static tare : Constant  Value=round((((1+p.accel.scaleError)*(cos(p.uncertainty.accelFrameAngle_rad)*(p.mechanics.gravity*sin(p.mechanics.angle))-sin(p.uncertainty.accelFrameAngle_rad)*(p.d.g))))/p.accel.quantum)*p.accel.quantum
  X new sample weight : Gain  Gain=1-exp(-p.sensor.sampleTime/p.accel.filterTime)
  X noisy sensor : Sum  Inputs=+++
  X old sample weight : Gain  Gain=exp(-p.sensor.sampleTime/p.accel.filterTime)
  X raw noise : RandomNumber  Seed=p.sensor.seed+336  SampleTime=p.sensor.sampleTime
  X raw noise RMS : Gain  Gain=p.adcStudy.d.accelerationNoiseInputRms_m_s2
  X select identified sensor response : Switch  Threshold=.5  SaturateOnIntegerOverflow=off  InputSameDT=off
  X sensor sampling : ZeroOrderHold  SampleTime=p.sensor.sampleTime
  X sensor scale : Gain  Gain=1+p.accel.scaleError
  X specific acceleration : Sum
  X tared acceleration : Sum  Inputs=+-
  X unknown drift : Sum
  X use engineered acquisition : Constant  Value=double(p.acquisition.enabled)
  Z ADC quantization : Quantizer  QuantizationInterval=1e-15
  Z acceleration range : Saturate  UpperLimit=inf  LowerLimit=-inf
  Z analog vibration probe : Sin  Amplitude=p.adcStudy.accelerationZAnalogToneAmplitude_m_s2  Frequency=2*pi*p.adcStudy.analogToneFrequency_Hz  Phase=p.adcStudy.analogTonePhase_rad  SampleTime=0
  Z drift after tare : Constant  Value=p.accel.bias
  Z engineered common AA and EMA : Subsystem
  Z filter memory : UnitDelay  InitialCondition=(1+p.accel.scaleError)*(cos(p.uncertainty.accelFrameAngle_rad)*(p.d.g)+sin(p.uncertainty.accelFrameAngle_rad)*(p.mechanics.gravity*sin(p.mechanics.angle)))  SampleTime=p.sensor.sampleTime
  Z fresh 10 kHz acceleration frame : ZeroOrderHold  SampleTime=p.force.sampleTime
  Z gravity : Constant  Value=p.d.g
  Z identified sensor response : Sum
  Z known channel delay : TransportDelay  DelayTime=p.adcStudy.d.channels.acceleration.pipelineDelay_s  InitialOutput=p.accel.bias
  Z known static tare : Constant  Value=round((((1+p.accel.scaleError)*(cos(p.uncertainty.accelFrameAngle_rad)*(p.d.g)+sin(p.uncertainty.accelFrameAngle_rad)*(p.mechanics.gravity*sin(p.mechanics.angle)))))/p.accel.quantum)*p.accel.quantum
  Z new sample weight : Gain  Gain=1-exp(-p.sensor.sampleTime/p.accel.filterTime)
  Z noisy sensor : Sum  Inputs=+++
  Z old sample weight : Gain  Gain=exp(-p.sensor.sampleTime/p.accel.filterTime)
  Z raw noise : RandomNumber  Seed=p.sensor.seed+239  SampleTime=p.sensor.sampleTime
  Z raw noise RMS : Gain  Gain=p.adcStudy.d.accelerationNoiseInputRms_m_s2
  Z select identified sensor response : Switch  Threshold=.5  SaturateOnIntegerOverflow=off  InputSameDT=off
  Z sensor sampling : ZeroOrderHold  SampleTime=p.sensor.sampleTime
  Z sensor scale : Gain  Gain=1+p.accel.scaleError
  Z specific acceleration : Sum
  Z tared acceleration : Sum  Inputs=+-
  Z unknown drift : Sum
  Z use engineered acquisition : Constant  Value=double(p.acquisition.enabled)
  tag scope: measured_S_acceleration_x=global, measured_S_acceleration_z=global, physical_S_acceleration_x=global, physical_S_acceleration_z=global
  wires:
  Physical S motion/1 -> Physical S acceleration Z/1
  Physical S acceleration Z/1 -> [physical_S_acceleration_z], Z specific acceleration/1
  Z gravity/1 -> Z specific acceleration/2
  Z sensor scale/1 -> Z sensor sampling/1, Z noisy sensor/1
  Z raw noise/1 -> Z raw noise RMS/1
  Z raw noise RMS/1 -> Z noisy sensor/2
  Z noisy sensor/1 -> Z new sample weight/1, Z engineered common AA and EMA/1(analog input)
  Z new sample weight/1 -> Z identified sensor response/1
  Z identified sensor response/1 -> Z filter memory/1, Z select identified sensor response/3
  Z filter memory/1 -> Z old sample weight/1
  Z old sample weight/1 -> Z identified sensor response/2
  Z acceleration range/1 -> Z ADC quantization/1
  Z ADC quantization/1 -> Z tared acceleration/1
  Z known static tare/1 -> Z tared acceleration/2
  Z tared acceleration/1 -> Z unknown drift/1
  Z drift after tare/1 -> Z unknown drift/2
  Physical S acceleration X/1 -> [physical_S_acceleration_x], X specific acceleration/1
  X gravity/1 -> X specific acceleration/2
  X specific acceleration/1 -> Acceleration Z frame cross axis/1, Acceleration X frame diagonal/1
  X sensor scale/1 -> X sensor sampling/1, X noisy sensor/1
  X raw noise/1 -> X raw noise RMS/1
  X raw noise RMS/1 -> X noisy sensor/2
  X noisy sensor/1 -> X new sample weight/1, X engineered common AA and EMA/1(analog input)
  X new sample weight/1 -> X identified sensor response/1
  X identified sensor response/1 -> X filter memory/1, X select identified sensor response/3
  X filter memory/1 -> X old sample weight/1
  X old sample weight/1 -> X identified sensor response/2
  X acceleration range/1 -> X ADC quantization/1
  X ADC quantization/1 -> X tared acceleration/1
  X known static tare/1 -> X tared acceleration/2
  X tared acceleration/1 -> X unknown drift/1
  X drift after tare/1 -> X unknown drift/2
  Z use engineered acquisition/1 -> Z select identified sensor response/2
  Z select identified sensor response/1 -> Z acceleration range/1
  Z fresh 10 kHz acceleration frame/1 -> [measured_S_acceleration_z]
  X use engineered acquisition/1 -> X select identified sensor response/2
  X select identified sensor response/1 -> X acceleration range/1
  X fresh 10 kHz acceleration frame/1 -> [measured_S_acceleration_x]
  Z specific acceleration/1 -> Acceleration Z frame diagonal/1, Acceleration X frame cross axis/1
  Acceleration Z frame diagonal/1 -> Acceleration Z frame calibrated sum/1
  Acceleration Z frame cross axis/1 -> Acceleration Z frame calibrated sum/2
  Acceleration Z frame calibrated sum/1 -> Z sensor scale/1
  Acceleration X frame diagonal/1 -> Acceleration X frame calibrated sum/1
  Acceleration X frame cross axis/1 -> Acceleration X frame calibrated sum/2
  Acceleration X frame calibrated sum/1 -> X sensor scale/1
  Z analog vibration probe/1 -> Z noisy sensor/3
  Z engineered common AA and EMA/1(conditioned output) -> Z select identified sensor response/1
  Z unknown drift/1 -> Z known channel delay/1
  Z known channel delay/1 -> Z fresh 10 kHz acceleration frame/1
  X analog vibration probe/1 -> X noisy sensor/3
  X engineered common AA and EMA/1(conditioned output) -> X select identified sensor response/1
  X unknown drift/1 -> X known channel delay/1
  X known channel delay/1 -> X fresh 10 kHz acceleration frame/1
